simulink model "Adaptive_Edge_Cloud_Simulation"  (R2026b)
settings: Solver=VariableStepAuto
settings Model: Creator=Siddhi  LastModifiedBy=Siddhi

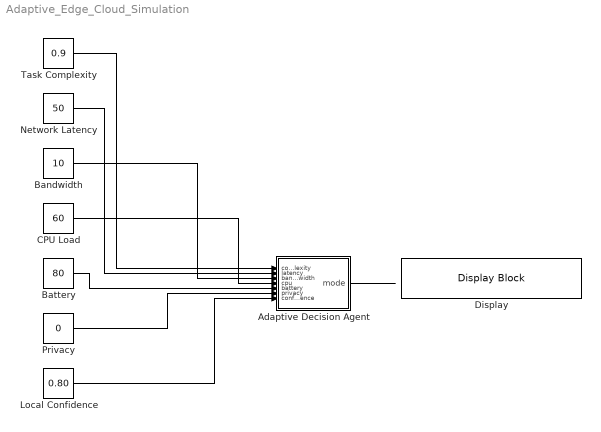
== system Adaptive_Edge_Cloud_Simulation ==
  Adaptive Decision Agent : MATLAB Function  TreatAsAtomicUnit=on
  Bandwidth : Constant  Value=10
  Battery : Constant  Value=80
  CPU Load : Constant  Value=60
  Display : DisplayBlock  LabelPosition=Hide  Transparency=1  GridColor=[0.502, 0.502, 0.502]
  Local Confidence : Constant  Value=0.80  VectorParams1D=off
  Network Latency : Constant  Value=50
  Privacy : Constant  Value=0
  Task Complexity : Constant  Value=0.9
  wires:
  Task Complexity/1 -> Adaptive Decision Agent/1(complexity)
  Network Latency/1 -> Adaptive Decision Agent/2(latency)
  Bandwidth/1 -> Adaptive Decision Agent/3(bandwidth)
  CPU Load/1 -> Adaptive Decision Agent/4(cpu)
  Battery/1 -> Adaptive Decision Agent/5(battery)
  Privacy/1 -> Adaptive Decision Agent/6(privacy)
  Local Confidence/1 -> Adaptive Decision Agent/7(confidence)
  Adaptive Decision Agent/1(mode) -> ?

== matlab function Adaptive_Edge_Cloud_Simulation/Adaptive Decision Agent ==
  data: complexity input; mode output; latency input; bandwidth input; cpu input; battery input; privacy input; confidence input
function mode = adaptiveAgent(complexity, latency, bandwidth, cpu, battery, privacy, confidence)
%#codegen

% 1 = EDGE
% 2 = HYBRID
% 3 = CLOUD

if privacy == 1
    mode = 1;

elseif latency > 180 || bandwidth < 3
    mode = 1;

elseif confidence < 0.65
    mode = 2;

elseif complexity > 0.75 && latency < 100
    mode = 3;

elseif cpu > 80 && latency < 100
    mode = 3;

elseif battery < 20 && latency < 100
    mode = 3;

else
    mode = 1;
end
